simulink model "sim_aug"  (R2026a)
settings: Solver=VariableStepAuto  StopTime=40
values from neighbouring files (symbols this model uses):
  batt = struct()    [init_params.m]
  drone = struct()    [init_params.m]
  SoC0 = 1    [init_params.m]
  w0_motor = mot.w_h.*ones(4,1)    [init_params.m]
  xi0 = [0;0;0]    [init_params.m]
undefined symbols (not defined in the file or in its folder): mot
libraries: matrix_library x1, slpidlib x1
settings Model: Creator=flow  LastModifiedBy=flow

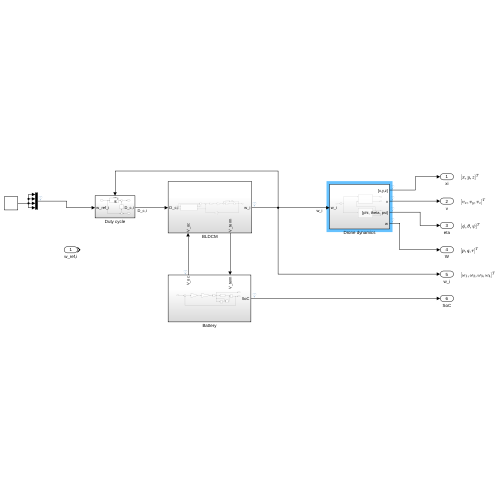
[thumbnail: Simulink's stored preview of the top-level diagram]
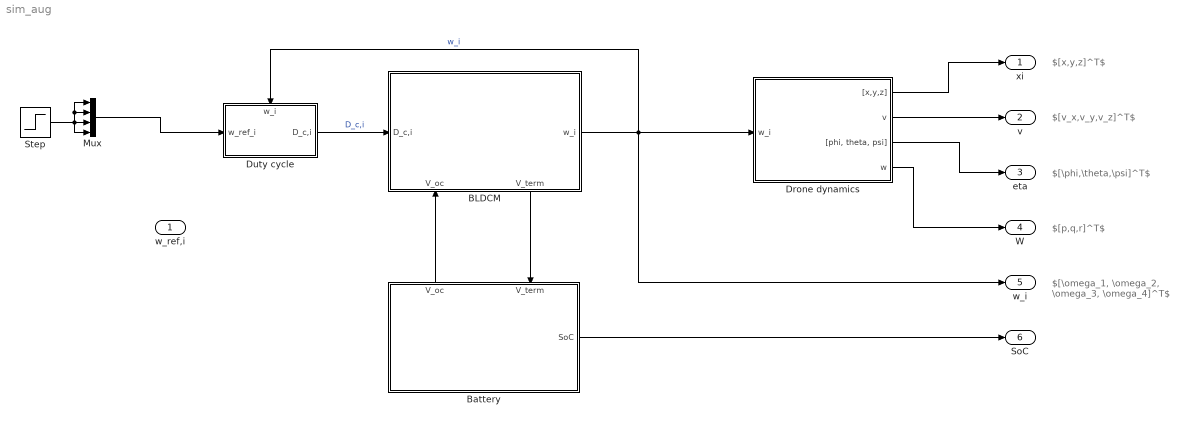
== system sim_aug ==
  note: $[x,y,z]^T$
  note: $[v_x,v_y,v_z]^T$
  note: $[\phi,\theta,\psi]^T$
  note: $[p,q,r]^T$
  note: $[\omega_1, \omega_2, \omega_3, \omega_4]^T$
  w_ref,i : Inport  PortDimensions=4
  BLDCM : Subsystem
      settings: PortSchema="{\"entries\":[{\"content\":{\"sides\":[{\"content\":{\"connectorIds\":[\"In1\"]},\"type\":\"ConnectorPlacement.EquallySpacedRectSide\",\"uuid\":\"afaeb7da-edbb-4bca-a60b-399a137f3982\"},{\"content\":{\"connectorIds\":[\"Out1\"],\"side\":\"RIGHT\"},\"type\":\"ConnectorPlacement.EquallySpacedRectSide\",\"uuid\":\"5bacb964-0447-466a-8069-01888f805414\"},{\"content\":{\"side\":\"TOP\"},\"type\":\"ConnectorPlacement.EquallySpacedRectSide\",\"uuid\":\"bae93f6c-ee08-4660-ad29-e4dc824a3145\"},{\"content\":{\"connectorIds\":[\"In2\",\"Out2\"],\"side\":\"BOTTOM\"},\"type\":\"ConnectorPlacement.EquallySpacedRectSide\",\"uuid\":\"35edff43-7f1d-4fe5-9bcc-f2e383a66153\"}]},\"type\":\"ConnectorPlacement.EquallySpacedConnector\",\"uuid\":\"1f5c3918-7770-48ce-8888-918caa1fa4a1\"}],\"packageUris\":[\"http://schema.mathworks.com/mf0/Connector/R2020b\"],\"version\":\"1.0\"}"
  Battery : Subsystem
      settings: PortSchema="{\"entries\":[{\"content\":{\"sides\":[{\"content\":{},\"type\":\"ConnectorPlacement.EquallySpacedRectSide\",\"uuid\":\"e6822eb3-bd33-48a1-81cc-b0fb141b0ba1\"},{\"content\":{\"connectorIds\":[\"Out1\"],\"side\":\"RIGHT\"},\"type\":\"ConnectorPlacement.EquallySpacedRectSide\",\"uuid\":\"d837e6ba-e606-41d2-886b-21dc98ed8dda\"},{\"content\":{\"connectorIds\":[\"Out2\",\"In1\"],\"side\":\"TOP\"},\"type\":\"ConnectorPlacement.EquallySpacedRectSide\",\"uuid\":\"1d25bf0a-f5cc-4267-a4a1-4a52a94e30fd\"}]},\"type\":\"ConnectorPlacement.EquallySpacedConnector\",\"uuid\":\"5ffb67be-acea-4381-815d-570dafeb1c70\"}],\"packageUris\":[\"http://schema.mathworks.com/mf0/Connector/R2020b\"],\"version\":\"1.0\"}"
  Drone dynamics : Subsystem
  Duty cycle : Subsystem
      settings: PortSchema="{\"entries\":[{\"content\":{\"sides\":[{\"content\":{\"connectorIds\":[\"In1\"]},\"type\":\"ConnectorPlacement.EquallySpacedRectSide\",\"uuid\":\"eb071dd1-afc4-4573-98b2-06372cbb1b03\"},{\"content\":{\"connectorIds\":[\"Out1\"],\"side\":\"RIGHT\"},\"type\":\"ConnectorPlacement.EquallySpacedRectSide\",\"uuid\":\"f955facd-bc02-4912-9630-31e84e18e9d5\"},{\"content\":{\"connectorIds\":[\"In2\"],\"side\":\"TOP\"},\"type\":\"ConnectorPlacement.EquallySpacedRectSide\",\"uuid\":\"f8ec3f30-b72a-40e7-b617-6a93d3e6c80c\"}]},\"type\":\"ConnectorPlacement.EquallySpacedConnector\",\"uuid\":\"8bfdd951-2858-48aa-8462-5ae76b5f6b80\"}],\"packageUris\":[\"http://schema.mathworks.com/mf0/Connector/R2020b\"],\"version\":\"1.0\"}"
  Mux : Mux
  Step : Step  Time=15  InitialValue=0.9*drone.w_h  FinalValue=1.1*drone.w_h  SampleTime=0
  xi : Outport
  v : Outport  Port=2
  eta : Outport  Port=3
  W : Outport  Port=4
  w_i : Outport  Port=5
  SoC : Outport  Port=6
  wires:
  Battery/2(V_oc) -> BLDCM/2(V_oc)
  BLDCM/2(V_term) -> Battery/1(V_term)
  Duty cycle/1(D_c,i) -> BLDCM/1(D_c,i)  "D_c,i"
  BLDCM/1(w_i) -> Drone dynamics/1(w_i), w_i/1, Duty cycle/2(w_i)  "w_i"
  Drone dynamics/1("[x,y,z]") -> xi/1
  Drone dynamics/2(v) -> v/1
  Drone dynamics/3("[phi, theta, psi]") -> eta/1
  Drone dynamics/4(w) -> W/1
  Battery/1(SoC) -> SoC/1
  Step/1 -> Mux/1, Mux/2, Mux/3, Mux/4
  Mux/1 -> Duty cycle/1(w_ref_i)

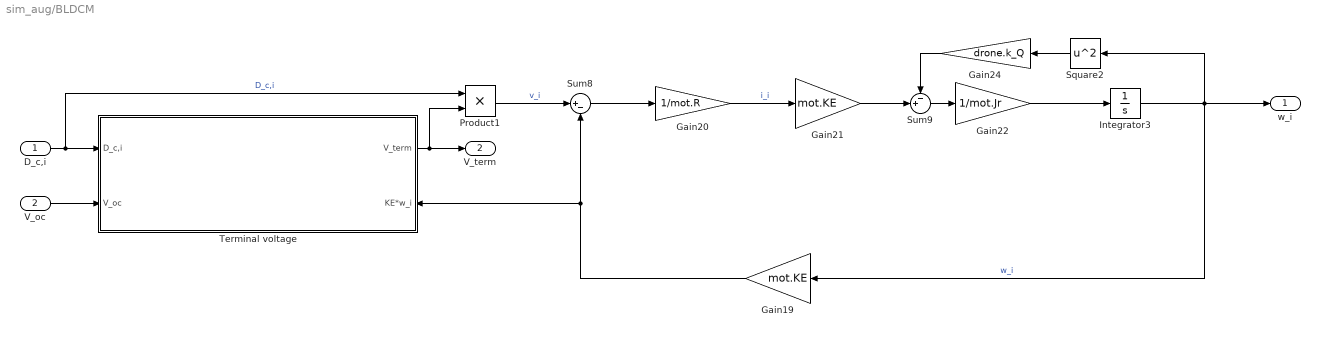
== system sim_aug/BLDCM ==
  D_c,i : Inport
  V_oc : Inport  Port=2
  Gain19 : Gain  Gain=mot.KE
  Gain20 : Gain  Gain=1/mot.R
  Gain21 : Gain  Gain=mot.KE
  Gain22 : Gain  Gain=1/mot.Jr
  Gain24 : Gain  Gain=drone.k_Q
  Integrator3 : Integrator  InitialCondition=w0_motor
  Product1 : Product
  Square2 : Math  Operator=square
  Sum8 : Sum  Inputs=|+-
  Sum9 : Sum  Inputs=-+|
  Terminal voltage : Subsystem
      settings: PortSchema="{\"entries\":[{\"content\":{\"sides\":[{\"content\":{\"connectorIds\":[\"In1\",\"In2\"]},\"type\":\"ConnectorPlacement.EquallySpacedRectSide\",\"uuid\":\"6ec7c31c-9b49-4c5d-a004-0a6df891eb05\"},{\"content\":{\"connectorIds\":[\"Out1\",\"In3\"],\"side\":\"RIGHT\"},\"type\":\"ConnectorPlacement.EquallySpacedRectSide\",\"uuid\":\"5e82088f-3817-4311-908c-0e8efc9bebc9\"},{\"content\":{\"side\":\"TOP\"},\"type\":\"ConnectorPlacement.EquallySpacedRectSide\",\"uuid\":\"cf387629-afa3-4fd0-8f4d-44df74a131e4\"}]},\"type\":\"ConnectorPlacement.EquallySpacedConnector\",\"uuid\":\"e7135423-0c01-4a6f-9161-d20c526d0bb5\"}],\"packageUris\":[\"http://schema.mathworks.com/mf0/Connector/R2020b\"],\"version\":\"1.0\"}"
  w_i : Outport
  V_term : Outport  Port=2
  wires:
  Sum8/1 -> Gain20/1
  Integrator3/1 -> Square2/1, w_i/1, Gain19/1  "w_i"
  Product1/1 -> Sum8/1  "v_i"
  Square2/1 -> Gain24/1
  Gain21/1 -> Sum9/2
  D_c,i/1 -> Product1/1, Terminal voltage/1(D_c,i)  "D_c,i"
  Gain20/1 -> Gain21/1  "i_i"
  Sum9/1 -> Gain22/1
  Gain22/1 -> Integrator3/1
  Gain19/1 -> Terminal voltage/3(KE*w_i), Sum8/2
  Gain24/1 -> Sum9/1
  V_oc/1 -> Terminal voltage/2(V_oc)
  Terminal voltage/1(V_term) -> V_term/1, Product1/2

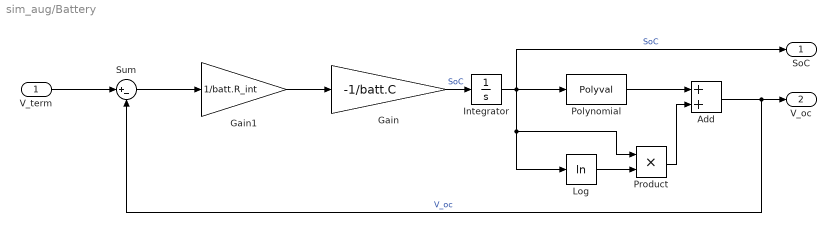
== system sim_aug/Battery ==
  V_term : Inport
  Add : Sum
  Gain : Gain  Gain=-1/batt.C
  Gain1 : Gain  Gain=1/batt.R_int
  Integrator : Integrator  InitialCondition=SoC0
  Log : Math  Operator=log
  Polynomial : Polyval  Coefs=batt.Pol_ocv
  Product : Product
  Sum : Sum  Inputs=|+-
  SoC : Outport
  V_oc : Outport  Port=2
  wires:
  Gain/1 -> Integrator/1  "SoC"
  Add/1 -> Sum/2, V_oc/1  "V_oc"
  Product/1 -> Add/2
  Log/1 -> Product/2
  Integrator/1 -> Polynomial/1, Log/1, Product/1, SoC/1  "SoC"
  Polynomial/1 -> Add/1
  V_term/1 -> Sum/1
  Sum/1 -> Gain1/1
  Gain1/1 -> Gain/1

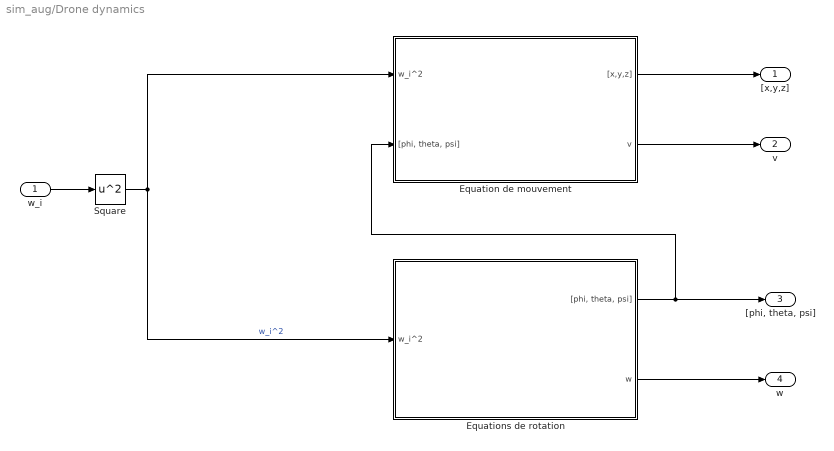
== system sim_aug/Drone dynamics ==
  w_i : Inport
  Equation de mouvement : Subsystem
  Equations de rotation : Subsystem
  Square : Math  Operator=square
  "[x,y,z]" : Outport
  v : Outport  Port=2
  "[phi, theta, psi]" : Outport  Port=3
  w : Outport  Port=4
  wires:
  Square/1 -> Equations de rotation/1(w_i^2), Equation de mouvement/1(w_i^2)  "w_i^2"
  Equation de mouvement/1("[x,y,z]") -> "[x,y,z]"/1
  Equation de mouvement/2(v) -> v/1
  Equations de rotation/1("[phi, theta, psi]") -> "[phi, theta, psi]"/1, Equation de mouvement/2("[phi, theta, psi]")
  Equations de rotation/2(w) -> w/1
  w_i/1 -> Square/1

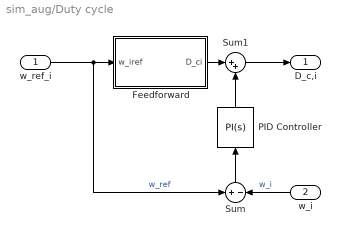
== system sim_aug/Duty cycle ==
  w_ref_i : Inport
  w_i : Inport  Port=2
  Feedforward : Subsystem
  PID Controller : slpidlib/PID Controller  Controller=PI  Form=Parallel  TimeDomain=Continuous-time  UseExternalTs=off  SampleTime=-1  IntegratorMethod=Forward Euler  FilterMethod=Forward Euler  ControllerParametersSource=internal  P=9.4e-4  I=9.42e-2  UseKiTs=off  D=0  UseExternalDerivativeSource=off  N=100  UseFilter=on  TunerSelectOption=Transfer Function Based (PID Tuner App)  InitialConditionSource=internal  InitialConditionForIntegrator=0  InitialConditionForFilter=0  DifferentiatorICPrevScaledInput=0  ExternalReset=none  TrackingMode=off  Kt=1  LimitOutput=off  SatLimitsSource=internal  UpperSaturationLimit=inf  LowerSaturationLimit=-inf  LinearizeAsGain=on  AntiWindupMode=none  Kb=1  LimitIntegrator=off  UpperIntegratorSaturationLimit=inf  LowerIntegratorSaturationLimit=-inf  POutMin=[]  POutMax=[]  IOutMin=[]  IOutMax=[]  DOutMin=[]  DOutMax=[]  NOutMin=[]  NOutMax=[]  SumOutMin=[]  SumOutMax=[]  SaturationOutMin=[]  SaturationOutMax=[]  PParamMin=[]  PParamMax=[]  IParamMin=[]  IParamMax=[]  DParamMin=[]  DParamMax=[]  NParamMin=[]  NParamMax=[]  KbParamMin=[]  KbParamMax=[]  KtParamMin=[]  KtParamMax=[]  KbOutMin=[]  KbOutMax=[]  KtOutMin=[]  KtOutMax=[]  IntegratorOutMin=[]  IntegratorOutMax=[]  FilterOutMin=[]  FilterOutMax=[]  SumI1OutMin=[]  SumI1OutMax=[]  SumI2OutMin=[]  SumI2OutMax=[]  SumI3OutMin=[]  SumI3OutMax=[]  SumI4OutMin=[]  SumI4OutMax=[]  SumDOutMin=[]  SumDOutMax=[]  DifferentiatorOutMin=[]  DifferentiatorOutMax=[]  FilterDiffOutCoefMin=[]  FilterDiffOutCoefMax=[]  ReciprocalOutMin=[]  ReciprocalOutMax=[]  SumDenOutMin=[]  SumDenOutMax=[]  SumNumOutMin=[]  SumNumOutMax=[]  DivideOutMin=[]  DivideOutMax=[]  UdiffTsProdOutMin=[]  UdiffTsProdOutMax=[]  NTsProdOutMin=[]  NTsProdOutMax=[]  UintegralTsProdOutMin=[]  UintegralTsProdOutMax=[]  UngainTsProdOutMin=[]  UngainTsProdOutMax=[]  ClampingZeroOutDataTypeStr=Inherit: Inherit via back propagation  ClampingZeroOutMin=[]  ClampingZeroOutMax=[]  FilterDenConstantOutDataTypeStr=Inherit: Inherit via back propagation  FilterDenConstantOutMin=[]  FilterDenConstantOutMax=[]  PCopyOutDataTypeStr=Inherit: Inherit via back propagation  PCopyOutMin=[]  PCopyOutMax=[]  NCopyOutDataTypeStr=Inherit: Inherit via back propagation  NCopyOutMin=[]  NCopyOutMax=[]  IntegratorContinuousStateAttributes=''  IntegratorStateMustResolveToSignalObject=off  IntegratorRTWStateStorageClass=Auto  FilterContinuousStateAttributes=''  FilterStateMustResolveToSignalObject=off  FilterRTWStateStorageClass=Auto  ParallelPVariant=InternalParameters  IdealPVariant=Disabled  IVariant=InternalParameters  DVariant=Disabled  IntegratorVariant=Continuous  SatVariant=Disabled  AWVariant=Passthrough  PCopyVariant=Disabled  TRVariant=Disabled  FdbkBlocksVariant=Forward  IdealPFdbkVariant=Disabled  SatFdbkVariant=Disabled  DerivativeFilterVariant=Disabled  NVariant=Disabled  NCopyVariant=Disabled_SignalSpec  FilterICVariant=Disabled  IntegratorICVariant=InternalICs  ExternalResetVariant=Disabled  TRSumVariant=Passthrough  SumFdbkVariant=Disabled  SumVariant=Sum_PI  TsampFilterVariant=InternalTs  TsampNgainVariant=Passthrough  TsampIntegralVariant=Disabled_SignalSpec  ExternalSaturationOutDataTypeStr=Inherit: Same as second input  DerivativeSourceVariant=Disabled  PreIntVariant=InternalPreInt
  Sum : Sum  Inputs=+|-
  Sum1 : Sum  Inputs=|++
  D_c,i : Outport
  wires:
  w_ref_i/1 -> Sum/1, Feedforward/1(w_iref)  "w_ref"
  PID Controller/1 -> Sum1/2
  Sum/1 -> PID Controller/1
  w_i/1 -> Sum/2  "w_i"
  Sum1/1 -> D_c,i/1
  Feedforward/1(D_ci) -> Sum1/1

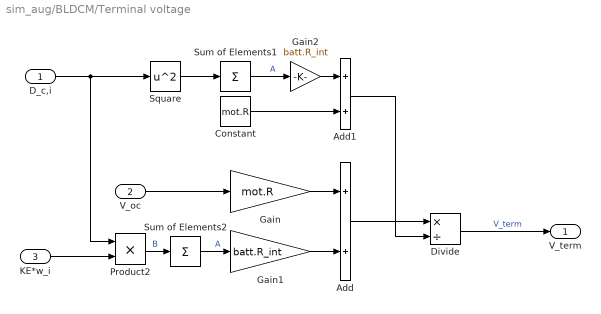
== system sim_aug/BLDCM/Terminal voltage ==
  D_c,i : Inport
  V_oc : Inport  Port=2
  KE*w_i : Inport  Port=3
  Add : Sum
  Add1 : Sum
  Constant : Constant  Value=mot.R
  Divide : Product  Inputs=*/
  Gain : Gain  Gain=mot.R
  Gain1 : Gain  Gain=batt.R_int
  Gain2 : Gain  Gain=batt.R_int
  Product2 : Product
  Square : Math  Operator=square
  Sum of Elements1 : Sum  Inputs=+
  Sum of Elements2 : Sum  Inputs=+
  V_term : Outport
  wires:
  Add/1 -> Divide/1
  Gain2/1 -> Add1/1
  Add1/1 -> Divide/2
  Gain/1 -> Add/1
  Product2/1 -> Sum of Elements2/1  "B"
  V_oc/1 -> Gain/1
  Gain1/1 -> Add/2
  KE*w_i/1 -> Product2/2
  Constant/1 -> Add1/2
  Square/1 -> Sum of Elements1/1
  Sum of Elements1/1 -> Gain2/1  "A"
  D_c,i/1 -> Square/1, Product2/1
  Divide/1 -> V_term/1  "V_term"
  Sum of Elements2/1 -> Gain1/1  "A"

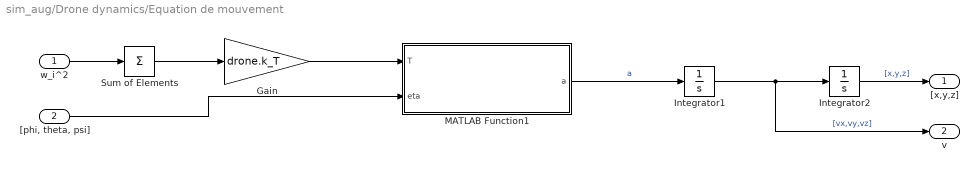
== system sim_aug/Drone dynamics/Equation de mouvement ==
  w_i^2 : Inport
  "[phi, theta, psi]" : Inport  Port=2
  Gain : Gain  Gain=drone.k_T
  Integrator1 : Integrator
  Integrator2 : Integrator  InitialCondition=xi0
  MATLAB Function1 : MATLAB Function  TreatAsAtomicUnit=on
  Sum of Elements : Sum  Inputs=+
  "[x,y,z]" : Outport
  v : Outport  Port=2
  wires:
  MATLAB Function1/1(a) -> Integrator1/1  "a"
  Integrator1/1 -> v/1, Integrator2/1  "[vx,vy,vz]"
  Gain/1 -> MATLAB Function1/1(T)
  Sum of Elements/1 -> Gain/1
  Integrator2/1 -> "[x,y,z]"/1  "[x,y,z]"
  w_i^2/1 -> Sum of Elements/1
  "[phi, theta, psi]"/1 -> MATLAB Function1/2(eta)

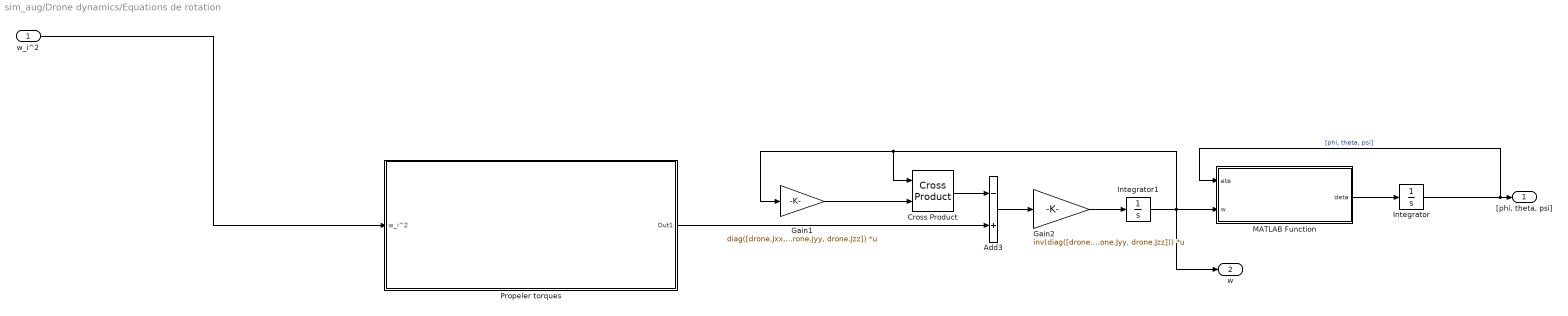
== system sim_aug/Drone dynamics/Equations de rotation ==
  w_i^2 : Inport
  Add3 : Sum  Inputs=-+
  Cross Product : matrix_library/Cross Product
  Gain1 : Gain  Gain=diag([drone.Jxx, drone.Jyy, drone.Jzz])  Multiplication=Matrix(K*u) (u vector)
  Gain2 : Gain  Gain=inv(diag([drone.Jxx, drone.Jyy, drone.Jzz]))  Multiplication=Matrix(K*u) (u vector)
  Integrator : Integrator
  Integrator1 : Integrator
  MATLAB Function : MATLAB Function  TreatAsAtomicUnit=on
  Propeler torques : Subsystem
  "[phi, theta, psi]" : Outport
  w : Outport  Port=2
  wires:
  MATLAB Function/1(deta) -> Integrator/1
  Add3/1 -> Gain2/1
  w_i^2/1 -> Propeler torques/1(w_i^2)
  Gain1/1 -> Cross Product/2
  Cross Product/1 -> Add3/1
  Propeler torques/1(Out1) -> Add3/2
  Integrator/1 -> MATLAB Function/1(eta), "[phi, theta, psi]"/1  "[phi, theta, psi]"
  Gain2/1 -> Integrator1/1
  Integrator1/1 -> w/1, Gain1/1, Cross Product/1, MATLAB Function/2(w)

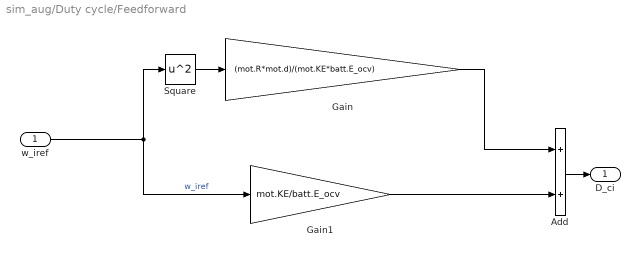
== system sim_aug/Duty cycle/Feedforward ==
  w_iref : Inport
  Add : Sum
  Gain : Gain  Gain=(mot.R*mot.d)/(mot.KE*batt.E_ocv)
  Gain1 : Gain  Gain=mot.KE/batt.E_ocv
  Square : Math  Operator=square
  D_ci : Outport
  wires:
  Gain1/1 -> Add/2
  Add/1 -> D_ci/1
  Gain/1 -> Add/1
  w_iref/1 -> Gain1/1, Square/1  "w_iref"
  Square/1 -> Gain/1

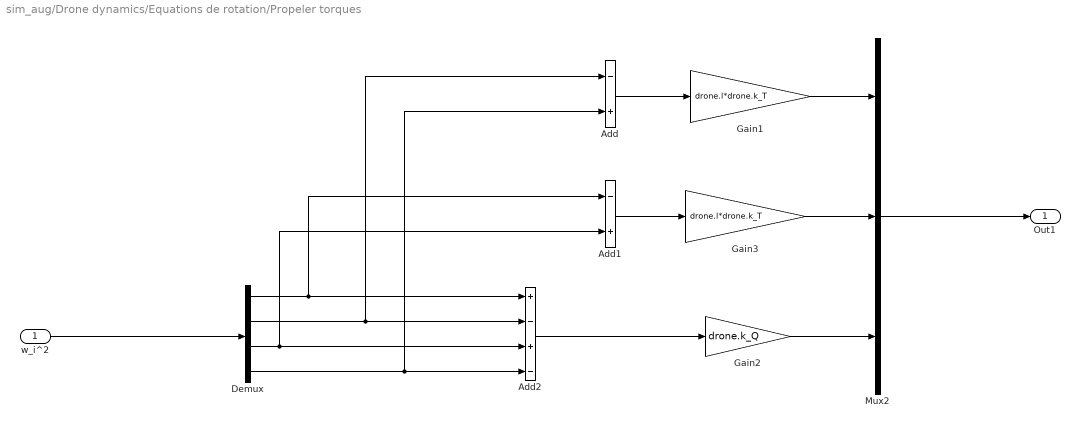
== system sim_aug/Drone dynamics/Equations de rotation/Propeler torques ==
  w_i^2 : Inport
  Add : Sum  Inputs=-+
  Add1 : Sum  Inputs=-+
  Add2 : Sum  Inputs=+-+-
  Demux : Demux
  Gain1 : Gain  Gain=drone.l*drone.k_T
  Gain2 : Gain  Gain=drone.k_Q
  Gain3 : Gain  Gain=drone.l*drone.k_T
  Mux2 : Mux  Inputs=3
  Out1 : Outport
  wires:
  Add1/1 -> Gain3/1
  Demux/3 -> Add2/3, Add1/2
  Gain2/1 -> Mux2/3
  Demux/4 -> Add2/4, Add/2
  Gain3/1 -> Mux2/2
  w_i^2/1 -> Demux/1
  Demux/1 -> Add2/1, Add1/1
  Mux2/1 -> Out1/1
  Add2/1 -> Gain2/1
  Demux/2 -> Add2/2, Add/1
  Add/1 -> Gain1/1
  Gain1/1 -> Mux2/1

== matlab function sim_aug/Drone dynamics/Equations de rotation/MATLAB Function ==
  data: eta input size=[3 1]; deta output size=[3 1]; w input size=[3 1]
function deta = fcn(eta,w)

phi = eta(1);
theta = eta(2);
psi = eta(3);

cphi    = cos(phi);
sphi    = sin(phi);
ctheta  = cos(theta);
stheta  = sin(theta);
ttheta  = stheta/ctheta;
cpsi    = cos(psi);
spsi    = sin(psi);



% Matrice de dérivation des angles d'euler
W = [1  sphi*ttheta cphi*ttheta;
    0  cphi        -sphi;
    0  sphi/ctheta cphi/ctheta];

% eta = [phi; theta; psi]
deta = W*w;

== matlab function sim_aug/Drone dynamics/Equation de mouvement/MATLAB Function1 ==
  data: T input size=1; a output size=[3 1]; eta input size=[3 1]
function a = fcn(T, eta)

m = 0.5;
g = 9.81;

phi = eta(1);
theta = eta(2);
psi = eta(3);

cphi    = cos(phi);
sphi    = sin(phi);
ctheta  = cos(theta);
stheta  = sin(theta);
cpsi    = cos(psi);
spsi    = sin(psi);

% Matrice de transition du repère du quadroptere dans le repere
% terrestre
R = [cpsi*ctheta,  cpsi*stheta*sphi - spsi*cphi,  cpsi*stheta*cphi + spsi*sphi;
    spsi*ctheta,  spsi*stheta*sphi + cpsi*cphi,  spsi*stheta*cphi - cpsi*sphi;
    -stheta,      ctheta*sphi,                   ctheta*cphi];

a = (1/m)*(R*[0;0;T]-[0;0;m*g]);
